simulink model "RL_dataCollection_v1"  (R2025a)
settings: Solver=VariableStepAuto  StartTime=0.0  StopTime=625  RelTol=1e-3
undefined symbols (not defined in the file or in its folder): National_Instruments, PCI
libraries: sldrtlib x3
settings Model: Creator=dperera  LastModifiedBy=dperera

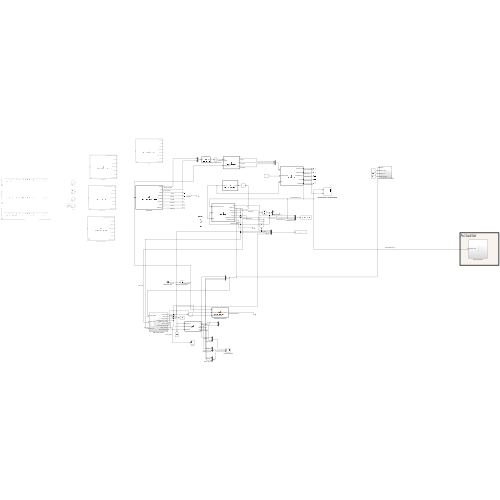
[thumbnail: Simulink's stored preview of the top-level diagram]
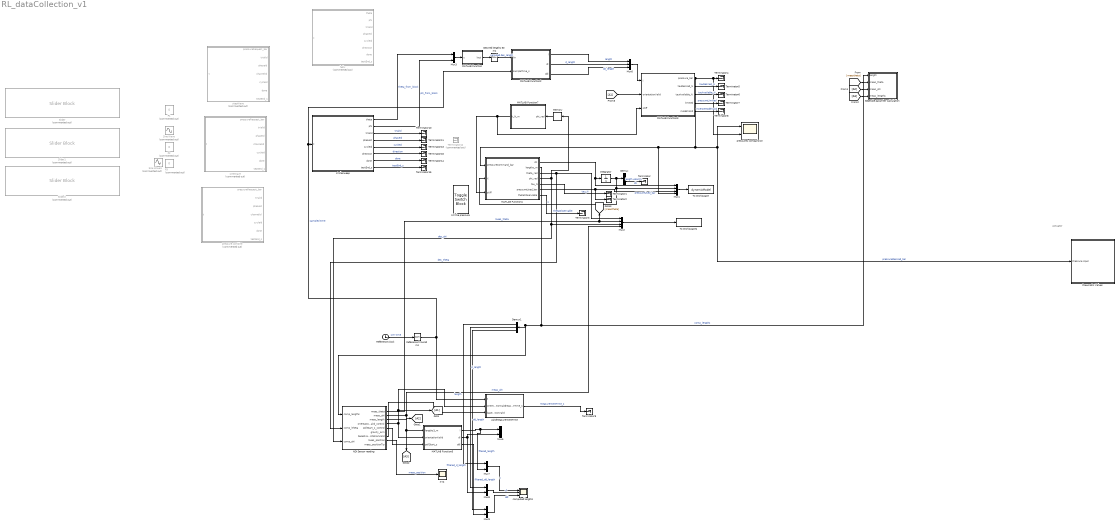
== system RL_dataCollection_v1 ==
  note: Actuator
  Demux : Demux  Outputs=2
  Demux1 : Demux  Outputs=3
  Desired lengths 50 ms : ZeroOrderHold  SampleTime=0.05
  Integrator : Integrator  InitialCondition=[0;0;0;0]
  MATLAB Function : MATLAB Function  TreatAsAtomicUnit=on
  MATLAB Function1 : MATLAB Function  TreatAsAtomicUnit=on
  MATLAB Function2 : MATLAB Function  TreatAsAtomicUnit=on
  MATLAB Function3 : MATLAB Function  TreatAsAtomicUnit=on
  MATLAB Function5 : MATLAB Function  TreatAsAtomicUnit=on
  MATLAB Function7 : MATLAB Function  TreatAsAtomicUnit=on
  Memory : Memory  InitialCondition=0.01
  Mux1 : Mux
  Mux2 : Mux
  Mux{3,5,7..9} (5 alike) : Mux  Inputs=2
  Mux6 : Mux  Inputs=3
  NDI Sensor reading : Subsystem
  P1 : Constant  Commented=on  Value=0
  P2 : Constant  Commented=on  Value=0
  P3 : Constant  Commented=on  Value=0
  Pneumatic Valves : Subsystem
  Reference clock : Clock
  Reference time 50 ms : ZeroOrderHold  SampleTime=0.05
  Seperate paramter calculation : Subsystem
  Sine Wave : Sin  Commented=on  Amplitude=1.5  Bias=1.5  Frequency=0.2  Phase=3*pi/2  SampleTime=0
  Sine Wave1 : Sin  Commented=on  Amplitude=1.5  Bias=1.5  Frequency=0.2  Phase=3*pi/2  SampleTime=0
  Slider : SliderBlock  Commented=on  ScaleMax=3
  Slider1 : SliderBlock  Commented=on  ScaleMax=3
  Slider2 : SliderBlock  Commented=on  ScaleMax=3
  Terminator{,1..11,13..16} (16 alike) : Terminator
  Terminator12 : Terminator  Commented=on
  To Workspace : ToWorkspace  VariableName=dynamicModel  SaveFormat=Timeseries  SampleTime=-1
  To Workspace1 : ToWorkspace  VariableName=dynamic_NDI_meas_angle  SaveFormat=Timeseries  SampleTime=-1
  XYZ : Scope
      settings: ActiveDisplayYMinimum=-0.091510816574096682  ActiveDisplayYMaximum=0.32359734916687011  DataLoggingVariableName=ScopeData15
  circlesweep : MATLAB Function  TreatAsAtomicUnit=on
  computed lengths : Scope  NumInputPorts=3
      settings: ActiveDisplayYMinimum=-0.016802180124961048  ActiveDisplayYMaximum=0.019521084576218834  DataLoggingVariableName=ScopeData11
  helix : MATLAB Function  Commented=on  TreatAsAtomicUnit=on
  kill the pressure : ToggleSwitchBlock
  pressure combine : MATLAB Function  Commented=on  TreatAsAtomicUnit=on
  pressures comparision : Scope  NumInputPorts=2
      settings: ActiveDisplayYMinimum=-0.2233120983765764  ActiveDisplayYMaximum=2.0098088853891882  DataLoggingVariableName=ScopeData6
  sineWave : MATLAB Function  Commented=on  TreatAsAtomicUnit=on
  stepWave : MATLAB Function  Commented=on  TreatAsAtomicUnit=on
  validMeasurementTime : MATLAB Function  TreatAsAtomicUnit=on
  wires:
  MATLAB Function1/1(dX) -> Mux1/1, Integrator/1  "dX"
  Integrator/1 -> MATLAB Function1/2(X), Mux1/2, Demux/1  "X"
  Demux/2 -> Terminator/1  "length velocity"
  MATLAB Function1/5(tau_N) -> Terminator1/1  "tau_N"
  MATLAB Function1/6(pressureUsed_bar) -> Terminator2/1, Mux1/3  "pressureUsed_bar"
  MATLAB Function1/7(thetaObservable) -> Terminator3/1  "thetaObservable"
  Mux1/1 -> To Workspace/1
  Mux2/1 -> To Workspace1/1
  Mux6/1 -> MATLAB Function3/1(l)
  [A1] -> MATLAB Function3/2(orientationValid)
  MATLAB Function3/1(pressure_bar) -> MATLAB Function1/1(pressureCommand_bar), Mux1/4, Pneumatic Valves/1(Pressure input), pressures comparision/1, pressures comparision/2, Terminator4/1  "pressureDesired_bar"
  MATLAB Function3/2(tauDesired_N) -> Terminator5/1  "tauDesired_N"
  MATLAB Function3/3(tauAvailable_N) -> Terminator6/1  "tauAvailable_N"
  MATLAB Function3/4(limited) -> Terminator7/1  "pressureLimited"
  MATLAB Function3/5(modelValid) -> Terminator8/1  "inverseModelValid"
  MATLAB Function7/1(k_N_m) -> MATLAB Function3/3(stiff), MATLAB Function1/3(stiff)
  Memory/1 -> MATLAB Function7/1(phi_rad)
  NDI Sensor reading/5(pollStart_s_control) -> MATLAB Function5/3(pollStart_s)
  NDI Sensor reading/8(meas_position) -> XYZ/1  "meas_position"
  MATLAB Function1/3(theta_rad) -> NDI Sensor reading/2(comp_ltheta), Mux2/1  "des_theta"
  NDI Sensor reading/1(meas_theta) -> [meastheta], Mux2/2  "meas_theta"
  NDI Sensor reading/3(meas_length) -> MATLAB Function5/1(lengths3_m), [A3]
  NDI Sensor reading/4(orientationValid_control) -> validMeasurementTime/2(orientationValid), [A1], MATLAB Function5/2(orientationValid)
  NDI Sensor reading/2(meas_phi) -> [A2], Mux2/4  "meas_phi"
  MATLAB Function5/1(l) -> Mux7/2, Mux5/1  "fitered_length"
  Demux1/3 -> Mux9/1  "dd_length"
  MATLAB Function1/4(phi_rad) -> NDI Sensor reading/3(comp_phi), Mux2/3, Memory/1  "des_phi"
  NDI Sensor reading/7(baseOreintationValid) -> validMeasurementTime/3(baseOrientationValid)
  Demux1/1 -> Mux7/1  "length"
  Demux1/2 -> Mux8/1  "d_length"
  Mux8/1 -> computed lengths/2  "dl"
  MATLAB Function5/3(ddl) -> Mux9/2  "filtered_dd_length"
  Mux7/1 -> computed lengths/1  "l"
  MATLAB Function5/2(dl) -> Mux8/2, Mux5/2  "filtered_d_length"
  Mux9/1 -> computed lengths/3  "ddl"
  [A3] -> Seperate paramter calculation/4(meas_lengths)
  [A2] -> Seperate paramter calculation/3(meas_phi)
  circlesweep/1(theta) -> Mux3/1  "theta_from_block"
  Reference clock/1 -> Reference time 50 ms/1  "sim time"
  Reference time 50 ms/1 -> circlesweep/1(t), MATLAB Function2/2(sampleTime_s), validMeasurementTime/1(t)  "sampled time"
  MATLAB Function1/2(lengths_m) -> Seperate paramter calculation/1(length), NDI Sensor reading/1(comp_lengths), Demux1/1  "comp_lengths"
  validMeasurementTime/1(measurementTime_s) -> Terminator9/1  "measurementTime_s"
  circlesweep/3(trialId) -> Terminator10/1  "trialId"
  circlesweep/4(phaseId) -> Terminator11/1  "phaseId"
  ? -> Terminator12/1  "channelId"
  circlesweep/5(cycleId) -> Terminator13/1  "cycleId"
  circlesweep/7(done) -> Terminator14/1  "done"
  circlesweep/8(testEnd_s) -> Terminator15/1  "testEnd_s"
  circlesweep/6(direction) -> Terminator16/1  "direction"
  MATLAB Function/1(lout) -> Desired lengths 50 ms/1
  Desired lengths 50 ms/1 -> MATLAB Function2/1(lIn)  "sampled des_length"
  Mux3/1 -> MATLAB Function/1(u)
  circlesweep/2(phi) -> Mux3/2  "phi_from_block"
  MATLAB Function2/1(l) -> Mux6/1  "length"
  MATLAB Function2/2(dl) -> Mux6/2  "d_length"
  MATLAB Function2/3(ddl) -> Mux6/3  "dd_length"
  [meastheta] -> Seperate paramter calculation/2(meas_theta)

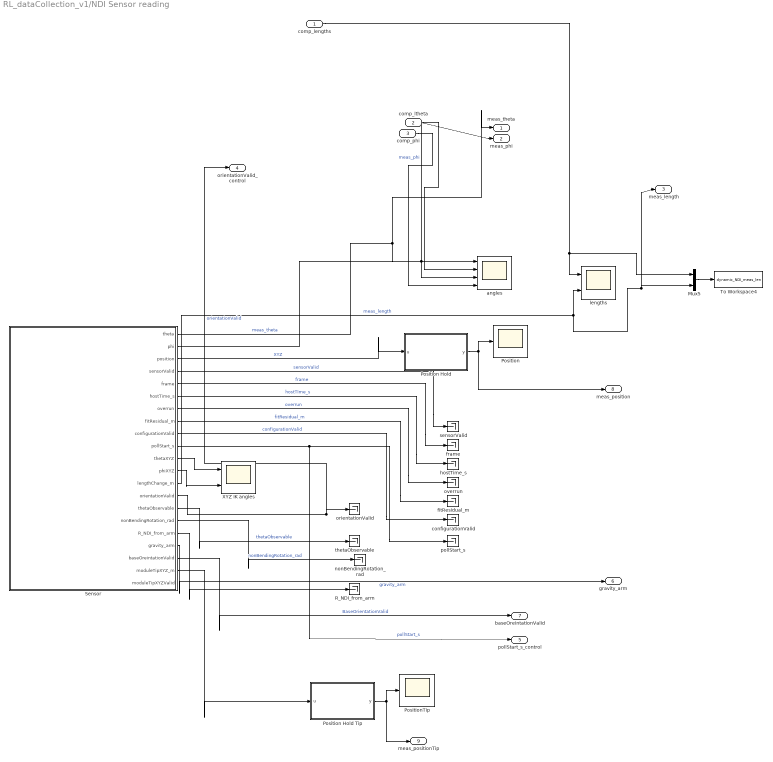
== system RL_dataCollection_v1/NDI Sensor reading ==
  comp_lengths : Inport
  comp_ltheta : Inport  Port=2
  comp_phi : Inport  Port=3
  Mux5 : Mux  Inputs=2
  Position : Scope
      settings: ActiveDisplayYMinimum=-0.21656345474719998  ActiveDisplayYMaximum=0.33777835857868188
  Position Hold : MATLAB Function  TreatAsAtomicUnit=on
  Position Hold Tip : MATLAB Function  TreatAsAtomicUnit=on
  PositionTip : Scope
      settings: ActiveDisplayYMinimum=-0.21656345474719998  ActiveDisplayYMaximum=0.33777835857868188  DataLoggingVariableName=ScopeData8
  R_NDI_from_arm : Terminator
  Sensor : Subsystem
  To Workspace4 : ToWorkspace  VariableName=dynamic_NDI_meas_len  SaveFormat=Timeseries  SampleTime=-1
  XYZ IK angles : Scope  NumInputPorts=2
      settings: DataLoggingVariableName=ScopeData2
  angles : Scope  NumInputPorts=4
      settings: ActiveDisplayYMinimum=-3.5335701463622691  ActiveDisplayYMaximum=3.3393501491613558
  configurationValid : Terminator
  fitResidual_m : Terminator
  frame : Terminator
  hostTime_s : Terminator
  lengths : Scope  NumInputPorts=2
      settings: ActiveDisplayYMinimum=-0.0017146774565175815  ActiveDisplayYMaximum=0.0020057370608089205  DataLoggingVariableName=ScopeData3
  nonBendingRotation_rad : Terminator
  orientationValid : Terminator
  overrun : Terminator
  pollStart_s : Terminator
  sensorValid : Terminator
  thetaObservable : Terminator
  meas_theta : Outport
  meas_phi : Outport  Port=2
  meas_length : Outport  Port=3
  orientationValid_control : Outport  Port=4
  pollStart_s_control : Outport  Port=5
  gravity_arm : Outport  Port=6
  baseOreintationValid : Outport  Port=7
  meas_position : Outport  Port=8
  meas_positionTip : Outport  Port=9
  wires:
  Sensor/13(lengthChange_m) -> lengths/2, meas_length/1, Mux5/2  "meas_length"
  comp_lengths/1 -> lengths/1, Mux5/1
  Sensor/10(pollStart_s) -> pollStart_s_control/1, pollStart_s/1  "pollStart_s"
  Sensor/2(phi) -> angles/3, meas_phi/1  "meas_phi"
  Sensor/3(position) -> Position Hold/1(u)  "XYZ"
  Sensor/1(theta) -> meas_theta/1, angles/1  "meas_theta"
  Sensor/6(hostTime_s) -> hostTime_s/1  "hostTIme_s"
  Sensor/9(configurationValid) -> configurationValid/1  "configurationValid"
  Sensor/4(sensorValid) -> sensorValid/1  "sensorValid"
  Sensor/7(overrun) -> overrun/1  "overrun"
  Sensor/5(frame) -> frame/1  "frame"
  comp_ltheta/1 -> angles/2
  Sensor/8(fitResidual_m) -> fitResidual_m/1  "fitResidual_m"
  Sensor/12(phiXYZ) -> XYZ IK angles/2
  Sensor/11(thetaXYZ) -> XYZ IK angles/1
  Position Hold/1(y) -> Position/1, meas_position/1
  Mux5/1 -> To Workspace4/1
  Sensor/14(orientationValid) -> orientationValid_control/1, orientationValid/1  "orientationValid"
  Sensor/16(nonBendingRotation_rad) -> nonBendingRotation_rad/1  "nonBendingRotation_rad"
  Sensor/15(thetaObservable) -> thetaObservable/1  "thetaObservable"
  comp_phi/1 -> angles/4
  Sensor/19(baseOreintationValid) -> baseOreintationValid/1  "BaseOrientationValid"
  Sensor/17(R_NDI_from_arm) -> R_NDI_from_arm/1
  Sensor/18(gravity_arm) -> gravity_arm/1  "gravity_arm"
  Sensor/20(moduleTipXYZ_m) -> Position Hold Tip/1(u)
  Position Hold Tip/1(y) -> meas_positionTip/1, PositionTip/1

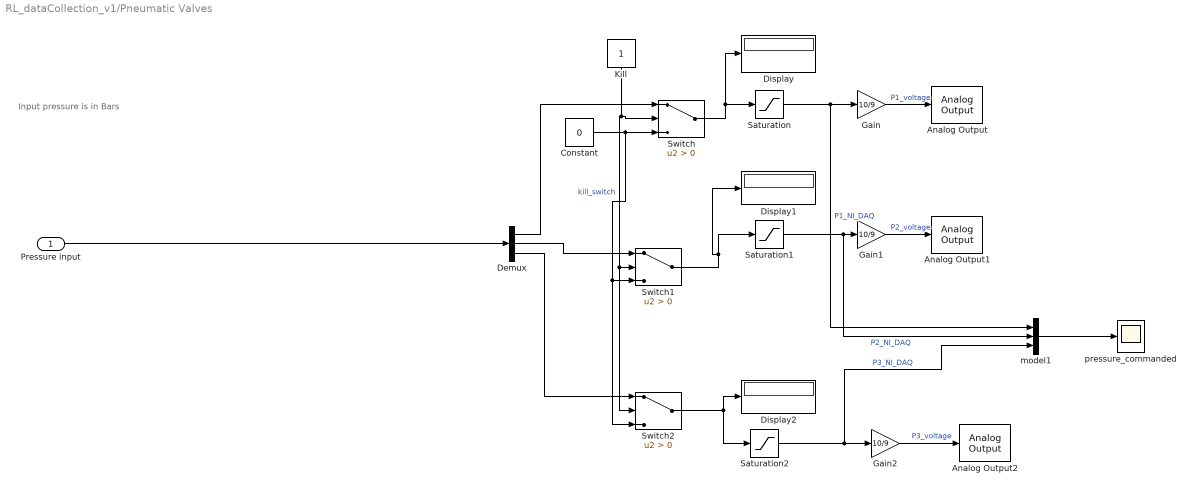
== system RL_dataCollection_v1/Pneumatic Valves ==
  note: Input pressure is in Bars
  Pressure input : Inport
  Analog Output : sldrtlib/Analog Output  SampleTime=1/100  MaxMissedTicks=inf  ShowMissedTicks=off  YieldWhenWaiting=off  DrvName=National_Instruments/PCI-6703  DrvAddress=4294967295  DrvOptions=0  Channels=1  RangeMode=1  VoltRange=1  InitialValue=0  FinalValue=0
      settings: AttributesFormatString=National Instruments\nPCI-6703 [auto]
  Analog Output1 : sldrtlib/Analog Output  SampleTime=1/100  MaxMissedTicks=inf  ShowMissedTicks=off  YieldWhenWaiting=off  DrvName=National_Instruments/PCI-6703  DrvAddress=4294967295  DrvOptions=0  Channels=2  RangeMode=1  VoltRange=1  InitialValue=0  FinalValue=0
      settings: AttributesFormatString=National Instruments\nPCI-6703 [auto]
  Analog Output2 : sldrtlib/Analog Output  SampleTime=1/100  MaxMissedTicks=inf  ShowMissedTicks=off  YieldWhenWaiting=off  DrvName=National_Instruments/PCI-6703  DrvAddress=4294967295  DrvOptions=0  Channels=3  RangeMode=1  VoltRange=1  InitialValue=0  FinalValue=0
      settings: AttributesFormatString=National Instruments\nPCI-6703 [auto]
  Constant : Constant  Value=0
  Demux : Demux  Outputs=3
  Display : Display
  Display1 : Display
  Display2 : Display
  Gain : Gain  Gain=10/9
  Gain1 : Gain  Gain=10/9
  Gain2 : Gain  Gain=10/9
  Kill : Constant
  Saturation : Saturate  UpperLimit=3  LowerLimit=0
  Saturation1 : Saturate  UpperLimit=3  LowerLimit=0
  Saturation2 : Saturate  UpperLimit=3  LowerLimit=0
  Switch : Switch  Criteria=u2 > Threshold  SaturateOnIntegerOverflow=off  InputSameDT=off
  Switch1 : Switch  Criteria=u2 > Threshold  SaturateOnIntegerOverflow=off  InputSameDT=off
  Switch2 : Switch  Criteria=u2 > Threshold  SaturateOnIntegerOverflow=off  InputSameDT=off
  model1 : Mux  Inputs=3
  pressure_commanded : Scope
      settings: ActiveDisplayYMinimum=-0.37499999999999989  ActiveDisplayYMaximum=3.375  DataLoggingVariableName=ScopeData7
  wires:
  Constant/1 -> Switch2/3, Switch1/3, Switch/3
  Kill/1 -> Switch2/2, Switch1/2, Switch/2  "kill_switch"
  Switch/1 -> Display/1, Saturation/1
  Gain/1 -> Analog Output/1  "P1_voltage"
  Saturation/1 -> model1/1, Gain/1  "P1_NI_DAQ"
  Demux/3 -> Switch2/1
  Gain1/1 -> Analog Output1/1  "P2_voltage"
  Gain2/1 -> Analog Output2/1  "P3_voltage"
  Saturation2/1 -> model1/3, Gain2/1  "P3_NI_DAQ"
  Switch2/1 -> Saturation2/1, Display2/1
  Demux/2 -> Switch1/1
  Switch1/1 -> Saturation1/1, Display1/1
  model1/1 -> pressure_commanded/1
  Saturation1/1 -> model1/2, Gain1/1  "P2_NI_DAQ"
  Demux/1 -> Switch/1
  Pressure input/1 -> Demux/1

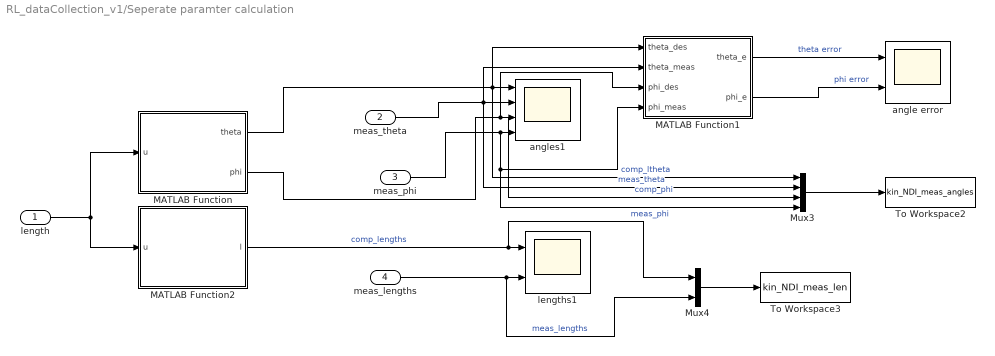
== system RL_dataCollection_v1/Seperate paramter calculation ==
  length : Inport
  meas_theta : Inport  Port=2
  meas_phi : Inport  Port=3
  meas_lengths : Inport  Port=4
  MATLAB Function : MATLAB Function  TreatAsAtomicUnit=on
  MATLAB Function1 : MATLAB Function  TreatAsAtomicUnit=on
  MATLAB Function2 : MATLAB Function  TreatAsAtomicUnit=on
  Mux3 : Mux
  Mux4 : Mux  Inputs=2
  To Workspace2 : ToWorkspace  VariableName=kin_NDI_meas_angles  SaveFormat=Timeseries  SampleTime=-1
  To Workspace3 : ToWorkspace  VariableName=kin_NDI_meas_len  SaveFormat=Timeseries  SampleTime=-1
  angle error : Scope  NumInputPorts=2
      settings: ActiveDisplayYMinimum=-3.908241267522468  ActiveDisplayYMaximum=3.9243412430226807  DataLoggingVariableName=ScopeData13
  angles1 : Scope  NumInputPorts=4
      settings: ActiveDisplayYMinimum=-3.9269137322662839  ActiveDisplayYMaximum=3.9265599408279468  DataLoggingVariableName=ScopeData4
  lengths1 : Scope  NumInputPorts=2
      settings: ActiveDisplayYMinimum=-0.02243223759551808  ActiveDisplayYMaximum=0.037530111947788623  DataLoggingVariableName=ScopeData5
  wires:
  meas_lengths/1 -> Mux4/2, lengths1/2  "meas_lengths"
  meas_theta/1 -> MATLAB Function1/2(theta_meas), Mux3/2, angles1/2  "meas_theta"
  MATLAB Function/2(phi) -> MATLAB Function1/3(phi_des), Mux3/3, angles1/3  "comp_phi"
  Mux3/1 -> To Workspace2/1
  meas_phi/1 -> MATLAB Function1/4(phi_meas), Mux3/4, angles1/4  "meas_phi"
  MATLAB Function/1(theta) -> MATLAB Function1/1(theta_des), Mux3/1, angles1/1  "comp_ltheta"
  Mux4/1 -> To Workspace3/1
  MATLAB Function2/1(l) -> Mux4/1, lengths1/1  "comp_lengths"
  length/1 -> MATLAB Function2/1(u), MATLAB Function/1(u)
  MATLAB Function1/1(theta_e) -> angle error/1  "theta error"
  MATLAB Function1/2(phi_e) -> angle error/2  "phi error"

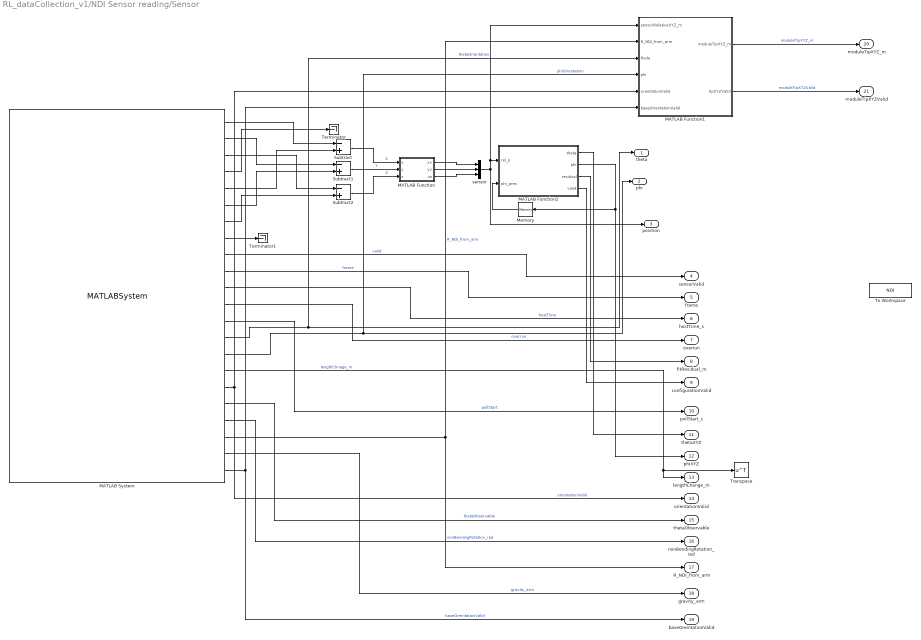
== system RL_dataCollection_v1/NDI Sensor reading/Sensor ==
  MATLAB Function : MATLAB Function  TreatAsAtomicUnit=on
  MATLAB Function1 : MATLAB Function  TreatAsAtomicUnit=on
  MATLAB Function2 : MATLAB Function  TreatAsAtomicUnit=on
  MATLAB System : MATLABSystem  System=AuroraReader_s2_BaseRotation  Port=COM12  BaudRate=921600  SamplePeriod=0.05  BaseSensorId=0A  TipSensorId=0B  CalibrationFile=C:\Users\dperera\OneDrive - Texas A&M University\Lab\Research\fDyn_ExpCom\hyDyn_Ctrl\ndi_orientation_recordings\calibration_20260930_190505_898.mat  PreflightSeconds=5  ActuatorRadius=0.013  ReferenceGravity_arm=[ 0; 0; -9.81 ]  SimulateUsing=Interpreted execution
      mask Type: AuroraReader_s2_BaseRotation
  Memory : Memory  InitialCondition=0.0001
  Subtract : Sum  Inputs=-+
  Subtract1 : Sum  Inputs=-+
  Subtract2 : Sum  Inputs=-+
  Terminator : Terminator
  Terminator1 : Terminator
  To Workspace : ToWorkspace  VariableName=NDI  SaveFormat=Timeseries  SampleTime=-1
  Transpose : Math  Operator=transpose
  sensor : Mux  Inputs=3
  theta : Outport
  phi : Outport  Port=2
  position : Outport  Port=3
  sensorValid : Outport  Port=4
  frame : Outport  Port=5
  hostTime_s : Outport  Port=6
  overrun : Outport  Port=7
  fitResidual_m : Outport  Port=8
  configurationValid : Outport  Port=9
  pollStart_s : Outport  Port=10
  thetaXYZ : Outport  Port=11
  phiXYZ : Outport  Port=12
  lengthChange_m : Outport  Port=13
  orientationValid : Outport  Port=14
  thetaObservable : Outport  Port=15
  nonBendingRotation_rad : Outport  Port=16
  R_NDI_from_arm : Outport  Port=17
  gravity_arm : Outport  Port=18
  baseOreintationValid : Outport  Port=19
  moduleTipXYZ_m : Outport  Port=20
  moduleTipXYZValid : Outport  Port=21
  wires:
  MATLAB System/2 -> Subtract1/1
  MATLAB Function/3(zz) -> sensor/3
  Subtract1/1 -> MATLAB Function/2(y)  "Y"
  Subtract2/1 -> MATLAB Function/3(z)  "Z"
  MATLAB System/5 -> Subtract/2
  sensor/1 -> MATLAB Function1/1(sensorRelativeXYZ_m), MATLAB Function2/1(rel_p), position/1
  MATLAB System/8 -> Terminator1/1
  MATLAB Function/1(xx) -> sensor/1
  Subtract/1 -> MATLAB Function/1(x)  "X"
  MATLAB Function/2(yy) -> sensor/2
  MATLAB System/1 -> Subtract/1
  MATLAB Function2/2(phi) -> Memory/1, phiXYZ/1
  MATLAB System/7 -> Subtract2/2
  MATLAB System/4 -> Terminator/1
  MATLAB System/3 -> Subtract2/1
  MATLAB System/6 -> Subtract1/2
  Memory/1 -> MATLAB Function2/2(phi_prev)
  MATLAB System/9 -> sensorValid/1  "valid"
  MATLAB System/11 -> hostTime_s/1  "hostTime"
  MATLAB System/12 -> overrun/1  "overrun"
  MATLAB Function2/3(residual) -> fitResidual_m/1
  MATLAB Function2/4(valid) -> configurationValid/1
  MATLAB System/13 -> pollStart_s/1  "pollStart"
  MATLAB System/14 -> MATLAB Function1/3(theta), theta/1  "thetaOrientation"
  MATLAB System/15 -> MATLAB Function1/4(phi), phi/1  "phiOrientation"
  MATLAB Function2/1(theta) -> thetaXYZ/1
  MATLAB System/16 -> lengthChange_m/1, Transpose/1  "lengthChnage_m"
  MATLAB System/17 -> orientationValid/1, MATLAB Function1/5(orientationValid)  "orientationValid"
  MATLAB System/18 -> thetaObservable/1  "thetaObservable"
  MATLAB System/19 -> nonBendingRotation_rad/1  "nonBendingRotation_rad"
  MATLAB System/10 -> frame/1  "frame"
  MATLAB System/20 -> R_NDI_from_arm/1, MATLAB Function1/2(R_NDI_from_arm)  "R_NDI_from_arm"
  MATLAB System/21 -> gravity_arm/1  "gravity_arm"
  MATLAB System/22 -> baseOreintationValid/1, MATLAB Function1/6(baseOrientationValid)  "baseOreintationValid"
  MATLAB Function1/1(moduleTipXYZ_m) -> moduleTipXYZ_m/1  "moduleTipXYZ_m"
  MATLAB Function1/2(tipXYZValid) -> moduleTipXYZValid/1  "moduleTipXYZValid"

== matlab function RL_dataCollection_v1/validMeasurementTime ==
  data: t input; measurementTime_s output; orientationValid input; baseOrientationValid input
function measurementTime_s = validMeasurementTime( ...
    t, orientationValid, baseOrientationValid)
%#codegen

persistent lastValidTime
if isempty(lastValidTime)
    lastValidTime = -1.0;
end

if orientationValid && baseOrientationValid && isfinite(t)
    lastValidTime = t;
end

measurementTime_s = lastValidTime;
end

== matlab function RL_dataCollection_v1/NDI Sensor reading/Position Hold Tip ==
  data: u input; y output
function y = fcn(u)
persistent lastPosition
if isempty(lastPosition), lastPosition=nan(3,1); end
if all(isfinite(u)), lastPosition=u; end
y=lastPosition;
end

== matlab function RL_dataCollection_v1/MATLAB Function5 ==
  data: lengths3_m input; l output; dl output; ddl output; orientationValid input; pollStart_s input
function [l, dl, ddl] = filteredDerivatives(lengths3_m, orientationValid, pollStart_s)
%#codegen
% NDI lengths are [l1;l2;l3]; model coordinates are [l2;l3].
% Invalid or repeated BX frames do not update the derivative states.
persistent lastL lastT velocity acceleration
if isempty(lastT)
    lastL = nan(2,1);
    lastT = -1;
    velocity = zeros(2,1);
    acceleration = zeros(2,1);
end
l = lastL;
dl = velocity;
ddl = acceleration;
if ~orientationValid || ~all(isfinite(lengths3_m)) || ~isfinite(pollStart_s)
    return;
end
q = [lengths3_m(2); lengths3_m(3)];
if lastT < 0
    lastL = q;
    lastT = pollStart_s;
    l = q;
    return;
end
dt = pollStart_s-lastT;
if dt > 1e-6
    rawVelocity = (q-lastL)/dt;
    oldVelocity = velocity;
    alphaV = dt/(0.20+dt);
    velocity = velocity + alphaV*(rawVelocity-velocity);
    rawAcceleration = (velocity-oldVelocity)/dt;
    alphaA = dt/(0.30+dt);
    acceleration = acceleration + alphaA*(rawAcceleration-acceleration);
    lastL = q;
    lastT = pollStart_s;
end
l = lastL;
dl = velocity;
ddl = acceleration;
end

== matlab function RL_dataCollection_v1/sineWave ==
  data: t input; pressureRequest_bar output; trialId output; phaseId output; channelId output; cycleId output; done output; testEnd_s output
function [pressureRequest_bar,trialId,phaseId,channelId,cycleId,done,testEnd_s] = rlPressureSineBlock(t)
%#codegen
% OPEN-LOOP raw pressure request: peak/2*(1-cos(omega*time)).
% channelSelection: 1=P1, 2=P2, 3=P3, 0=all three separately.
channelSelection=0;
peak_bar=3.0;
omega_radPerS=0.2;
cyclesPerTrial=3;
repeats=2;
initialZero_s=5.0;
relax_s=10.0;
% phase: -1 invalid time, 0 initial zero, 4 zero relaxation,
% 5 periodic excitation, 9 complete. Cycles join at zero with zero slope.
assert(channelSelection>=0 && channelSelection<=3 && channelSelection==floor(channelSelection));
assert(peak_bar>=0 && peak_bar<=3 && omega_radPerS>0);
assert(cyclesPerTrial>=1 && cyclesPerTrial==floor(cyclesPerTrial));
assert(repeats>=1 && repeats==floor(repeats) && initialZero_s>=0 && relax_s>0);
nChannels=1;if channelSelection==0,nChannels=3;end
period_s=2*pi/omega_radPerS;
excitation_s=cyclesPerTrial*period_s;
trialDuration_s=excitation_s+relax_s;
nTrials=nChannels*repeats;
testEnd_s=initialZero_s+nTrials*trialDuration_s;
pressureRequest_bar=zeros(3,1);trialId=0;phaseId=0;channelId=0;cycleId=0;done=false;
if ~isfinite(t) || t<0,phaseId=-1;return;end
if t<initialZero_s,return;end
if t>=testEnd_s,phaseId=9;done=true;return;end
index=floor((t-initialZero_s)/trialDuration_s);
trialId=index+1;channelId=channelSelection;
if channelSelection==0,channelId=floor(index/repeats)+1;end
local=t-initialZero_s-index*trialDuration_s;
if local<excitation_s
    phaseId=5;cycleId=floor(local/period_s)+1;
    pressureRequest_bar(channelId)=peak_bar*.5*(1-cos(omega_radPerS*local));
else
    phaseId=4;
end
end

== matlab function RL_dataCollection_v1/MATLAB Function7 ==
  data: phi_rad input; k_N_m output
function k_N_m = stiffnessFromPhiBlock(phi_rad)
%#codegen
% Scalar P1 effective stiffness from the 2026-10-02 fitted data (N/m).
% Input may be current phi or externally delayed phi, in radians.
% Endpoint extension: <=0.09425 rad -> 4132; >=2.05594 rad -> 953.333.
% Invalid input uses the near-straight endpoint (not a sensor-validity gate).
breaks = [0.094252336020426999 0.31719551885716302 ...
          0.84254655402063705 1.3628983100343199 ...
          1.7568402609821301 2.0559364288348001];
coefs = [-301.18295127845971 -90.779050026315701 -3508.295263988015 4132; ...
          8648.306884889811 -4672.8276757423591 -3593.6820922138418 3342; ...
          222.76060985869111 882.71017208803505 -1342.7968944369923 1418.3333333333301; ...
          341.14621515352195 107.09908322703643 -243.20935379879649 990; ...
          254.06580436465293 166.20780898136815 0 931.66666666666697];
if ~isfinite(phi_rad) || phi_rad <= breaks(1)
    k_N_m = 4132;
    return;
end
if phi_rad >= breaks(6)
    k_N_m = 953.333333333333;
    return;
end
segment = 1;
for j = 2:5
    if phi_rad >= breaks(j), segment = j; end
end
x = phi_rad-breaks(segment);
k_N_m = ((coefs(segment,1)*x+coefs(segment,2))*x ...
           +coefs(segment,3))*x+coefs(segment,4);
end

== matlab function RL_dataCollection_v1/stepWave ==
  data: t input; pressureRequest_bar output; trialId output; phaseId output; channelId output; cycleId output; done output; testEnd_s output
function [pressureRequest_bar,trialId,phaseId,channelId,cycleId,done,testEnd_s] = rlPressureStepsBlock(t)
%#codegen
% OPEN-LOOP REQUEST ONLY. Connect through the existing Kill/pressure limits.
% channelSelection: 1=P1, 2=P2, 3=P3, 0=all three tested separately.
channelSelection=0;
peakLevels_bar=[1.0 2.0 3.0];
repeats=2;
initialZero_s=5.0;
rise_s=5.0;
hold_s=10.0;
fall_s=5.0;
relax_s=10.0;
% phase: -1 invalid time, 0 initial zero, 1 rise, 2 hold, 3 fall,
% 4 zero relaxation, 9 complete. No deadzone subtraction.
assert(channelSelection>=0 && channelSelection<=3 && channelSelection==floor(channelSelection));
assert(repeats>=1 && repeats==floor(repeats));
assert(all(peakLevels_bar>=0 & peakLevels_bar<=3));
assert(initialZero_s>=0 && rise_s>0 && hold_s>0 && fall_s>0 && relax_s>0);
nChannels=1;if channelSelection==0,nChannels=3;end
nLevels=numel(peakLevels_bar);
trialDuration_s=rise_s+hold_s+fall_s+relax_s;
nTrials=nChannels*repeats*nLevels;
testEnd_s=initialZero_s+nTrials*trialDuration_s;
pressureRequest_bar=zeros(3,1);trialId=0;phaseId=0;channelId=0;cycleId=0;done=false;
if ~isfinite(t) || t<0,phaseId=-1;return;end
if t<initialZero_s,return;end
if t>=testEnd_s,phaseId=9;done=true;return;end
index=floor((t-initialZero_s)/trialDuration_s);
trialId=index+1;
channelId=channelSelection;
if channelSelection==0,channelId=floor(index/(repeats*nLevels))+1;end
cycleId=mod(floor(index/nLevels),repeats)+1;
level=mod(index,nLevels)+1;
local=t-initialZero_s-index*trialDuration_s;
peak=peakLevels_bar(level);
if local<rise_s
    phaseId=1;u=local/rise_s;p=peak*u*u*(3-2*u);
elseif local<rise_s+hold_s
    phaseId=2;p=peak;
elseif local<rise_s+hold_s+fall_s
    phaseId=3;u=(local-rise_s-hold_s)/fall_s;p=peak*(1-u*u*(3-2*u));
else
    phaseId=4;p=0;
end
pressureRequest_bar(channelId)=p;
end

== matlab function RL_dataCollection_v1/circlesweep ==
  data: t input; theta output; phi output; trialId output; phaseId output; cycleId output; direction output; done output; testEnd_s output
function [theta,phi,trialId,phaseId,cycleId,direction,done,testEnd_s] = rlCircleSweepReferenceBlock(t)
%#codegen
% Requested ANGLES, not pressures or measured arm motion.
% Five phi levels, five circles each, no pauses between revolutions.
phiLevels_rad=[0.2 0.8 1.0 1.2 1.5];
circleTime_s=20.0;
circlesPerTrial=5;
initialZero_s=5.0;
phiRise_s=5.0;
targetWait_s=3.0;
phiFall_s=5.0;
zeroHold_s=10.0;
rotationDirection=1; % +1 or -1; keep unwrapped theta for downstream rates.
% phase: -1 invalid,0 baseline,1 phi rise,2 target wait,3 phi fall,
% 4 zero hold,5 circles,9 complete.
assert(all(phiLevels_rad>=0 & phiLevels_rad<=pi));
assert(circleTime_s>0 && circlesPerTrial>=1 && circlesPerTrial==floor(circlesPerTrial));
assert(phiRise_s>0 && phiFall_s>0 && targetWait_s>=0 && zeroHold_s>=0 && initialZero_s>=0);
assert(abs(rotationDirection)==1);
circleDuration_s=circlesPerTrial*circleTime_s;
trialDuration_s=phiRise_s+targetWait_s+circleDuration_s+phiFall_s+zeroHold_s;
nTrials=numel(phiLevels_rad);
testEnd_s=initialZero_s+nTrials*trialDuration_s;
theta=0;phi=0;trialId=0;phaseId=0;cycleId=0;direction=0;done=false;
if ~isfinite(t) || t<0,phaseId=-1;return;end
if t<initialZero_s,return;end
if t>=testEnd_s
    theta=rotationDirection*2*pi*circlesPerTrial*nTrials;
    phaseId=9;done=true;return;
end
index=floor((t-initialZero_s)/trialDuration_s);
trialId=index+1;
local=t-initialZero_s-index*trialDuration_s;
targetPhi=phiLevels_rad(trialId);
thetaStart=rotationDirection*2*pi*circlesPerTrial*index;
theta=thetaStart;
circleStart=phiRise_s+targetWait_s;
circleEnd=circleStart+circleDuration_s;
if local<phiRise_s
    phaseId=1;u=local/phiRise_s;phi=targetPhi*u*u*(3-2*u);
elseif local<circleStart
    phaseId=2;phi=targetPhi;
elseif local<circleEnd
    phaseId=5;direction=rotationDirection;
    elapsed=local-circleStart;
    cycleId=floor(elapsed/circleTime_s)+1;
    theta=thetaStart+rotationDirection*2*pi*elapsed/circleTime_s;
    phi=targetPhi;
elseif local<circleEnd+phiFall_s
    phaseId=3;theta=thetaStart+rotationDirection*2*pi*circlesPerTrial;
    u=(local-circleEnd)/phiFall_s;phi=targetPhi*(1-u*u*(3-2*u));
else
    phaseId=4;theta=thetaStart+rotationDirection*2*pi*circlesPerTrial;
end
end

== matlab function RL_dataCollection_v1/Seperate paramter calculation/MATLAB Function1 ==
  data: theta_des input; theta_e output; phi_e output; theta_meas input; phi_des input; phi_meas input
function [theta_e, phi_e] = configError(theta_des, theta_meas, phi_des, phi_meas)
%#codegen
% This file computes wrapped theta and phi error
%
% Inputs:
%   theta_des   : desired theta [constant] (rad)
%   theta_meas  : measured theta [constant] (rad)
%   phi_des     : desired phi [constant] (rad)
%   phi_meas    : measured phi [constant] (rad)
%
% Outputs:
%   theta_e     : bending direction [constant] (rad)
%   phi_e       : bending amount [constant] (rad)

phi_e = phi_des - phi_meas;

delta_theta = theta_des - theta_meas;
theta_e = atan2(sin(delta_theta), cos(delta_theta));

end

== matlab function RL_dataCollection_v1/helix ==
  data: t input; theta output; phi output; trialId output; phaseId output; cycleId output; direction output; done output; testEnd_s output
function [theta,phi,trialId,phaseId,cycleId,direction,done,testEnd_s] = rlHelixReferenceBlock(t)
%#codegen
% Requested theta/phi: outward then inward spiral/helix-like arm-tip path.
% Actual XYZ follows arm geometry; this is not a constant-pitch Cartesian helix.
peakPhi_rad=1.5;
circleTime_s=20.0;
turnsLoading=3;
turnsUnloading=3;
numTrials=4;
initialZero_s=5.0;
zeroHold_s=10.0;
alternateDirection=true; % CW/CCW alternate BETWEEN trials, at phi=0.
% phase: -1 invalid,0 baseline,4 zero hold,6 loading helix,
% 7 unloading helix,9 complete. Rotation does not pause at maximum phi.
assert(peakPhi_rad>=0 && peakPhi_rad<=pi && circleTime_s>0);
assert(turnsLoading>=1 && turnsLoading==floor(turnsLoading));
assert(turnsUnloading>=1 && turnsUnloading==floor(turnsUnloading));
assert(numTrials>=1 && numTrials==floor(numTrials) && initialZero_s>=0 && zeroHold_s>=0);
loading_s=turnsLoading*circleTime_s;
unloading_s=turnsUnloading*circleTime_s;
moving_s=loading_s+unloading_s;
trialDuration_s=moving_s+zeroHold_s;
turnsTotal=turnsLoading+turnsUnloading;
testEnd_s=initialZero_s+numTrials*trialDuration_s;
theta=0;phi=0;trialId=0;phaseId=0;cycleId=0;direction=0;done=false;
if ~isfinite(t) || t<0,phaseId=-1;return;end
if t<initialZero_s,return;end
if t>=testEnd_s
    turnsAccumulated=turnsTotal*numTrials;
    if alternateDirection,turnsAccumulated=turnsTotal*mod(numTrials,2);end
    theta=2*pi*turnsAccumulated;phaseId=9;done=true;return;
end
index=floor((t-initialZero_s)/trialDuration_s);
trialId=index+1;local=t-initialZero_s-index*trialDuration_s;
rotationDirection=1;turnsBefore=turnsTotal*index;
if alternateDirection
    rotationDirection=1-2*mod(index,2);
    turnsBefore=turnsTotal*mod(index,2);
end
thetaStart=2*pi*turnsBefore;
theta=thetaStart+rotationDirection*2*pi*min(local,moving_s)/circleTime_s;
if local<loading_s
    phaseId=6;direction=rotationDirection;
    cycleId=floor(local/circleTime_s)+1;
    u=local/loading_s;phi=peakPhi_rad*u*u*(3-2*u);
elseif local<moving_s
    phaseId=7;direction=rotationDirection;
    cycleId=floor(local/circleTime_s)+1;
    u=(local-loading_s)/unloading_s;
    phi=peakPhi_rad*(1-u*u*(3-2*u));
else
    phaseId=4;
end
end

== matlab function RL_dataCollection_v1/MATLAB Function1 ==
  data: pressureCommand_bar input; X input; dX output; lengths_m output; theta_rad output; phi_rad output; tau_N output; pressureUsed_bar output; thetaObservable output; stiff input
% function dX  = DynamicModel(p, X)
%#codegen
% This file computes length velocity and accelration from pressures using the dynamic model.
%
% Inputs:
%   p   : pressures [3x1] (Pa)
%   X   : length derivatives [4x1] (m)
%         [l2; l3; dl2; dl3]
%
% Output:
%   dX  : length derivatives [4x1] (m)
%         [dl2; dl3; ddl2; ddl3]

function [dX, lengths_m, theta_rad, phi_rad, tau_N, ...
          pressureUsed_bar, thetaObservable] = forwardModel(pressureCommand_bar, X, stiff)
%#codegen
% pressureCommand_bar = [P1; P2; P3], nonnegative bar
% X = [l2; l3; dl2; dl3], with l1 = -l2-l3

L = 0.17411;
r = 0.013; % PMA radial offset from backbone (m)
mass = 0.1;
K = 650 * [2 1; 1 2];
% K = stiff * [2 1; 1 2];
D = 40 * eye(2);
gArm = [0; 0; -9.81];
mu = 2000;
lengthBounds = [-0.035; 0.035; 1e6];

pressureUsed_bar = min(max(pressureCommand_bar, 0), 3);
% pressureUsed_bar = max(min(max(pressureCommand_bar, 0), 3) - 0.8, 0);

pressureDiameter_m = 0.013; % Effective pressure-area diameter, independent of r
pressureRadius_m = pressureDiameter_m/2;
area = pi * pressureRadius_m^2;

% Positive P1, P2, P3 give the established -X, -60°, +60°
% nominal bending directions, respectively.
tau_N = area * 1e5 * [-1 1 0; -1 0 1] * pressureUsed_bar;

dX = armS_single_entry(0, X, L, r, mass, gArm, ...
                       K, D, tau_N, mu, lengthBounds);

l2 = X(1);
l3 = X(2);
lengths_m = [-l2-l3; l2; l3];

u = (l2+l3)/r;
v = (l3-l2)/(sqrt(3)*r);
phi_rad = hypot(u, v);
theta_rad = atan2(v, u);
thetaObservable = phi_rad > 0.5*pi/180;


end

== matlab function RL_dataCollection_v1/pressure combine ==
  data: t input; pressureRequest_bar output; trialId output; phaseId output; channelId output; cycleId output; done output; testEnd_s output
function [pressureRequest_bar,trialId,phaseId,channelId,cycleId,done,testEnd_s] = rlPressureCombinedBlock(t)
%#codegen
% OPEN-LOOP common/differential pressure excitation, not angle tracking.
% trialId: 1 common pulse, 2 symmetric s, 3 antisymmetric a, 4 rotating s/a.
% channelId=0 means combined channels. No deadzone compensation.
commonPeak_bar=2.0;
bias_bar=1.5;
differentialAmplitude_bar=0.5;
omega_radPerS=0.2;
cyclesPerTrial=2;
initialZero_s=5.0;
preloadRise_s=5.0;
preloadFall_s=5.0;
relax_s=10.0;
% phase: -1 invalid, 0 initial zero, 1 preload rise, 3 preload fall,
% 4 zero relaxation, 5 periodic excitation, 9 complete.
assert(commonPeak_bar>=0 && commonPeak_bar<=3 && differentialAmplitude_bar>=0);
% Conservative bound for the rotating differential combination.
assert(bias_bar-4*differentialAmplitude_bar/3>=0 && bias_bar+4*differentialAmplitude_bar/3<=3);
assert(omega_radPerS>0 && cyclesPerTrial>=1 && cyclesPerTrial==floor(cyclesPerTrial));
assert(initialZero_s>=0 && preloadRise_s>0 && preloadFall_s>0 && relax_s>0);
period_s=2*pi/omega_radPerS;
excitation_s=cyclesPerTrial*period_s;
trialDuration_s=preloadRise_s+excitation_s+preloadFall_s+relax_s;
testEnd_s=initialZero_s+4*trialDuration_s;
pressureRequest_bar=zeros(3,1);trialId=0;phaseId=0;channelId=0;cycleId=0;done=false;
if ~isfinite(t) || t<0,phaseId=-1;return;end
if t<initialZero_s,return;end
if t>=testEnd_s,phaseId=9;done=true;return;end
index=floor((t-initialZero_s)/trialDuration_s);trialId=index+1;
local=t-initialZero_s-index*trialDuration_s;
% Each mode has matching endpoints; preload/fall remove inter-mode jumps.
endpoint=zeros(3,1);
if trialId==2 || trialId==3,endpoint(:)=bias_bar;end
if trialId==4
    endpoint=[bias_bar-2*differentialAmplitude_bar/3; ...
        bias_bar+differentialAmplitude_bar/3;bias_bar+differentialAmplitude_bar/3];
end
if local<preloadRise_s
    phaseId=1;u=local/preloadRise_s;pressureRequest_bar=endpoint*u*u*(3-2*u);
elseif local<preloadRise_s+excitation_s
    phaseId=5;tau=local-preloadRise_s;angle=omega_radPerS*tau;
    cycleId=floor(tau/period_s)+1;
    if trialId==1
        pressureRequest_bar(:)=commonPeak_bar*.5*(1-cos(angle));
    else
        s=0;a=0;
        if trialId==2,s=differentialAmplitude_bar*sin(angle);end
        if trialId==3,a=differentialAmplitude_bar*sin(angle);end
        if trialId==4
            s=differentialAmplitude_bar*cos(angle);
            a=differentialAmplitude_bar*sin(angle);
        end
        pressureRequest_bar=[bias_bar-2*s/3;bias_bar+s/3-a;bias_bar+s/3+a];
    end
elseif local<preloadRise_s+excitation_s+preloadFall_s
    phaseId=3;u=(local-preloadRise_s-excitation_s)/preloadFall_s;
    pressureRequest_bar=endpoint*(1-u*u*(3-2*u));
else
    phaseId=4;
end
end

== matlab function RL_dataCollection_v1/MATLAB Function ==
  data: u input; lout output
function lout = config2length(u)
%#codegen
% Convert configuration variables to length changes
% Input (u):
%   u       : theta and phi [2x1] (rad)
%               theta angle (rad) [constant]
%               phi angle (rad) [constant]
%   r       : radial offset (m) [constant]
% 
% Output:
%   lout    : lenght changes (m) [s,1]


theta = u(1);
phi = u(2);
r = 0.013;

l = [-r * cos(theta) * phi;
    (0.5e0 * r * cos(theta) - sqrt(0.3e1) * r * sin(theta) / 0.2e1) * phi;
    (0.5e0 * r * cos(theta) + sqrt(0.3e1) * r * sin(theta) / 0.2e1) * phi];

lout = [l(2); l(3)];

end

== matlab function RL_dataCollection_v1/MATLAB Function2 ==
  data: lIn input; l output; dl output; ddl output; sampleTime_s input
function [l, dl, ddl] = lengthDerivatives(lIn, sampleTime_s)
%#codegen
% Desired reduced lengths [l2;l3] in m; derivatives in m/s and m/s^2.
% sampleTime_s is a 0.05 s zero-order-held Clock signal.
persistent lastL lastT velocity acceleration
if isempty(lastT)
    lastL = zeros(2,1);
    lastT = -1;
    velocity = zeros(2,1);
    acceleration = zeros(2,1);
end
l = lastL;
dl = velocity;
ddl = acceleration;
if ~all(isfinite(lIn)) || ~isfinite(sampleTime_s)
    return;
end
q = [lIn(1); lIn(2)];
if lastT < 0
    lastL = q;
    lastT = sampleTime_s;
    l = q;
    return;
end
dt = sampleTime_s - lastT;
if dt > 1e-6
    rawVelocity = (q-lastL)/dt;
    oldVelocity = velocity;
    alphaV = dt/(0.10+dt);
    velocity = velocity + alphaV*(rawVelocity-velocity);
    rawAcceleration = (velocity-oldVelocity)/dt;
    alphaA = dt/(0.15+dt);
    acceleration = acceleration + alphaA*(rawAcceleration-acceleration);
    lastL = q;
    lastT = sampleTime_s;
end
l = lastL;
dl = velocity;
ddl = acceleration;
end

== matlab function RL_dataCollection_v1/Seperate paramter calculation/MATLAB Function ==
  data: u input; theta output; phi output
function [theta, phi] = length2config(u)
%#codegen
% This file convert the length changes into theta/phi
%
% Inputs:
%   u       : length change[2x1] (m)
%             [l2; l3]
%
% Outputs:
%   theta   : bending direction [constant] (rad)
%   phi     : bending amount [constant] (rad)

l = [0.0; u(1); u(2)];
r  = 0.013;

c = [atan2(l(3) - l(2), sqrt(0.3e1) * (l(2) + l(3)));
    0.2e1 / 0.3e1 / r * sqrt((3 * l(2) ^ 2 + 3 * l(3) * l(2) + 3 * l(3) ^ 2))];

theta = c(1);
phi = c(2);

end

== matlab function RL_dataCollection_v1/Seperate paramter calculation/MATLAB Function2 ==
  data: u input; l output
function l = lengthVector(u)
%#codegen
% This file create the length vector
%
% Inputs:
%   u       : length change[2x1] (m)
%             [l2; l3]
%
% Outputs:
%   l   : bending direction [3x1] (m)

l = [-(u(1) + u(2)); u(1); u(2)];

end

== matlab function RL_dataCollection_v1/NDI Sensor reading/Position Hold ==
  data: u input; y output
function y = fcn(u)
persistent lastPosition
if isempty(lastPosition), lastPosition=nan(3,1); end
if all(isfinite(u)), lastPosition=u; end
y=lastPosition;
end

== matlab function RL_dataCollection_v1/NDI Sensor reading/Sensor/MATLAB Function ==
  data: x input; xx output; y input; z input; yy output; zz output
function [xx,yy,zz] = rotateX90(x,y,z)

    R = [1 0 0;
         0 0 1;
         0 -1 0];

    p = R*[x;y;z]*0.001;

    xx=p(1);
    yy=p(2);
    zz=p(3);

    
end

== matlab function RL_dataCollection_v1/NDI Sensor reading/Sensor/MATLAB Function2 ==
  data: rel_p input; theta output; phi output; phi_prev input; residual output; valid output
function [theta,phi,residual,valid] = xyz2ThetaPhi(rel_p,phi_prev)
persistent lastPhi lastTheta lastOutputTheta lastOutputPhi lastResidual
if isempty(lastPhi)
    lastPhi=0.0001; lastTheta=0;
    lastOutputTheta=NaN; lastOutputPhi=NaN; lastResidual=NaN;
end
% Keep the external memory for compatibility; never use its NaN.
if isfinite(phi_prev), lastPhi=phi_prev; end
[theta,phi,residual,valid]=ndiSupportFnc.configuration(rel_p,lastPhi,lastTheta);
if valid
    lastPhi=phi; lastTheta=theta;
    lastOutputTheta=theta; lastOutputPhi=phi; lastResidual=residual;
else
    % Scope outputs hold, but configurationValid remains false.
    theta=lastOutputTheta; phi=lastOutputPhi; residual=lastResidual;
end
end

== matlab function RL_dataCollection_v1/MATLAB Function3 ==
  data: l input; pressure_bar output; tauDesired_N output; tauAvailable_N output; limited output; modelValid output; orientationValid input; stiff input
function [pressure_bar, tauDesired_N, tauAvailable_N, limited, modelValid] = inverseModel(l, orientationValid, stiff)
%#codegen
% measured = [l2;l3;dl2;dl3;ddl2;ddl3] in SI units.
% Nonnegative pressure mapping uses the smallest common P1 pressure.

pressure_bar = zeros(3,1);
tauDesired_N = zeros(2,1);
tauAvailable_N = zeros(2,1);
limited = false;
modelValid = false;
if ~orientationValid || ~all(isfinite(l))
    return;
end
q = l(1:2);
dq = l(3:4);
ddq = l(5:6);
params.N = 1;
params.L = 0.17411;
params.r = 0.013;
params.mi = 0.1;
params.g = [0;0;-9.81];
params.K = 650*[2 1;1 2];
% params.K = stiff * [2 1; 1 2];
params.D = 40*eye(2);
params.mu = 2000;
params.lKbounds = [-0.035;0.035;1e6];
[M,C,G] = armS_single_core(q,dq,params);
Keff = params.K;
for i = 1:2
    Keff(i,i) = Keff(i,i) + 0.5*params.lKbounds(3)*(2 + ...
        tanh(params.mu*(q(i)-params.lKbounds(2))) - ...
        tanh(params.mu*(q(i)-params.lKbounds(1))));
end
tauDesired_N = M*ddq + (C+params.D)*dq + G + Keff*q;
if ~all(isfinite(tauDesired_N))
    tauDesired_N = zeros(2,1);
    return;
end
forcePerBar = pi*(params.r/2)^2*1e5;
forceBar = tauDesired_N/forcePerBar;
p1 = max([0;-forceBar(1);-forceBar(2)]);
effective = max([p1;p1+forceBar(1);p1+forceBar(2)],0);
deadzone_bar = 0.0;
maxCommand_bar = 3.0;
maxEffective_bar = maxCommand_bar-deadzone_bar;
peak = max(effective);
if peak > maxEffective_bar
    effective = effective*(maxEffective_bar/peak);
    limited = true;
end
for i = 1:3
    if effective(i) > 1e-8
        pressure_bar(i) = effective(i)+deadzone_bar;
    end
end
tauAvailable_N = forcePerBar*[-1 1 0;-1 0 1]*effective;
modelValid = true;
end

== matlab function RL_dataCollection_v1/NDI Sensor reading/Sensor/MATLAB Function1 ==
  data: sensorRelativeXYZ_m input; moduleTipXYZ_m output; R_NDI_from_arm input; theta input; phi input; orientationValid input; baseOrientationValid input; tipXYZValid output
function [moduleTipXYZ_m,tipXYZValid] = moduleTipXYZBlock( ...
    sensorRelativeXYZ_m,R_NDI_from_arm,theta,phi, ...
    orientationValid,baseOrientationValid)
%#codegen
% Input XYZ: existing Sensor/position output, metres, AFTER rotateX90.
% Output XYZ: physical module endpoint relative to module base, expressed
% in the CURRENT calibrated module-base frame. Not world-frame position.
% Assumes axial sensor mounting offsets: base .055 m, distal .050 m.
moduleTipXYZ_m=nan(3,1);
tipXYZValid=false;
if ~orientationValid || ~baseOrientationValid || ...
        ~all(isfinite(sensorRelativeXYZ_m(:))) || ...
        ~all(isfinite(R_NDI_from_arm(:))) || ...
        ~isfinite(theta) || ~isfinite(phi)
    return;
end
if norm(R_NDI_from_arm.'*R_NDI_from_arm-eye(3),'fro')>1e-3 || ...
        abs(det(R_NDI_from_arm)-1)>1e-3
    return;
end
% Undo the legacy fixed plotting-frame rotation, then use measured base pose.
R_fixed=[1 0 0;0 0 1;0 -1 0];
sensorXYZ_arm=R_NDI_from_arm.'*R_fixed.'*sensorRelativeXYZ_m(:);
% Measured tip tangent reconstructed from orientation-derived theta/phi.
% This does not reconstruct XYZ from a constant-curvature arc.
tipTangent=[sin(phi)*cos(theta);sin(phi)*sin(theta);cos(phi)];
moduleTipXYZ_m=sensorXYZ_arm-[0;0;0.055]-0.050*tipTangent;
tipXYZValid=true;
end
